simulink library "Simulation3DJoystickCalibratorLibrary"  (R2025b)
settings: Solver=VariableStepAuto  StartTime=0.0  StopTime=10.0  RelTol=1e-3
undefined symbols (not defined in the file or in its folder): aileronMax, aileronMin, elevatorMax, elevatorMin, helicopter, multirotor, pitchCh, pitchDB, pitchNeutral, rollCh, rollDB, rollNeutral, rudderMax, rudderMin, throttleCh, throttleDB, throttleMax, throttleMin, uPitchMax, uPitchMin, uRollMax, uRollMin, uThrottleMax, uThrottleMin, uYawMax, uYawMin, yawCh, yawDB, yawNeutral
libraries: sl3dlib x3
Description:
  | Simulation 3D Joystick Calibrator block library.
settings Model: Creator=klakhara  LastModifiedBy=klakhara

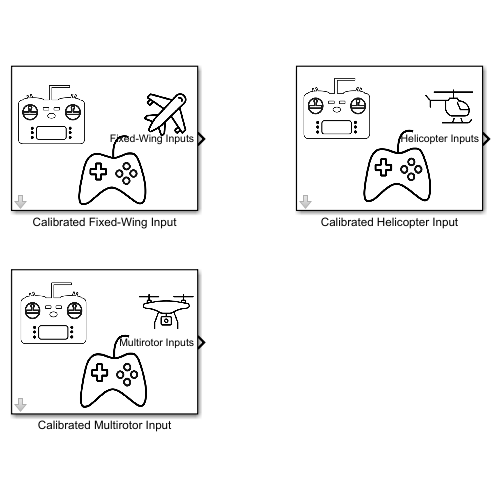
[thumbnail: Simulink's stored preview of the top-level diagram]
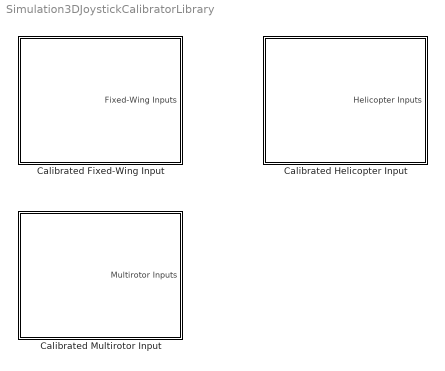
== system Simulation3DJoystickCalibratorLibrary ==
  Calibrated Fixed-Wing Input : Subsystem  mask{configName=0, joystickID=Joystick1, profileID=fixed-wing}
      mask prompts: joystickID "Device ID:"; profileID "Application profile"
      mask help: Calibrated Fixed-Wing Input. Accepts the shared Simulation 3D Joystick calibration. Output bus: Aileron, Elevator, Rudder, Throttle.
      mask TypeOptions joystickID: None | Joystick1 | Joystick2 | Joystick3 | Joystick4 | Joystick5 | Joystick6 | Joystick7 | Joystick8 | Joystick9 | Joystick10 | Joystick11 | Joystick12
      mask DialogControl DescGroupVar Prompt: Load Simulation 3D Joystick calibration
      mask DialogControl DescTextVar Prompt: Select a calibration configuration file:
      mask DialogControl loadConfig Prompt: Load file
      mask DialogControl openCalibrationApp Prompt: Open Calibration App
      mask DialogControl openCalibrationApp Tooltip: Open Simulation 3D Joystick Calibrator to create a calibration file.
      mask DialogControl ParameterGroupVar Prompt: Select the Simulation 3D Joystick device:
      mask Display: image('Calibrated Fixed Wing Aircraft Input.png');
  Calibrated Helicopter Input : Subsystem  mask{configName=0, joystickID=Joystick1, profileID=helicopter}
      mask prompts: joystickID "Device ID:"; profileID "Application profile"
      mask help: Calibrated Helicopter Input. Accepts the shared Simulation 3D Joystick calibration. Output bus: LateralCyclic, LongitudinalCyclic, Pedals, Collective.
      mask TypeOptions joystickID: None | Joystick1 | Joystick2 | Joystick3 | Joystick4 | Joystick5 | Joystick6 | Joystick7 | Joystick8 | Joystick9 | Joystick10 | Joystick11 | Joystick12
      mask DialogControl DescGroupVar Prompt: Load Simulation 3D Joystick calibration
      mask DialogControl DescTextVar Prompt: Select a calibration configuration file:
      mask DialogControl loadConfig Prompt: Load file
      mask DialogControl openCalibrationApp Prompt: Open Calibration App
      mask DialogControl openCalibrationApp Tooltip: Open Simulation 3D Joystick Calibrator to create a calibration file.
      mask DialogControl ParameterGroupVar Prompt: Select the Simulation 3D Joystick device:
      mask Display: image('Calibrated Helicopter Input.png');
  Calibrated Multirotor Input : Subsystem  mask{configName=0, joystickID=Joystick1, profileID=multirotor}
      mask prompts: joystickID "Device ID:"; profileID "Application profile"
      mask help: Calibrated Multirotor Input. Accepts the shared Simulation 3D Joystick calibration. Output bus: RollCmd, PitchCmd, YawCmd, ThrottleCmd.
      mask TypeOptions joystickID: None | Joystick1 | Joystick2 | Joystick3 | Joystick4 | Joystick5 | Joystick6 | Joystick7 | Joystick8 | Joystick9 | Joystick10 | Joystick11 | Joystick12
      mask DialogControl DescGroupVar Prompt: Load Simulation 3D Joystick calibration
      mask DialogControl DescTextVar Prompt: Select a calibration configuration file:
      mask DialogControl loadConfig Prompt: Load file
      mask DialogControl openCalibrationApp Prompt: Open Calibration App
      mask DialogControl openCalibrationApp Tooltip: Open Simulation 3D Joystick Calibrator to create a calibration file.
      mask DialogControl ParameterGroupVar Prompt: Select the Simulation 3D Joystick device:
      mask Display: image('Calibrated Rotorcraft Input.png');

== system Simulation3DJoystickCalibratorLibrary/Calibrated Fixed-Wing Input ==
  Actuator scaling : Subsystem
  CalibratedJoystickInput : BusCreator  Inputs=4
  Simulation 3D Joystick : sl3dlib/Simulation 3D/Hardware Interface/Simulation 3D Joystick  joyid=1  adjustports=on  forcefeed=off
  Terminator : Terminator
  Fixed-Wing Inputs : Outport
  wires:
  Simulation 3D Joystick/1 -> Actuator scaling/1(Raw Inputs)  "Raw Inputs"
  Actuator scaling/2(Elevator) -> CalibratedJoystickInput/2  "Elevator"
  Simulation 3D Joystick/2 -> Terminator/1
  CalibratedJoystickInput/1 -> Fixed-Wing Inputs/1  "Actuator deflections"
  Actuator scaling/3(Rudder) -> CalibratedJoystickInput/3  "Rudder"
  Actuator scaling/4(Throttle) -> CalibratedJoystickInput/4  "Throttle"
  Actuator scaling/1(Aileron) -> CalibratedJoystickInput/1  "Aileron"

== system Simulation3DJoystickCalibratorLibrary/Calibrated Helicopter Input ==
  Actuator scaling : Subsystem
  CalibratedJoystickInput : BusCreator  Inputs=4
  Simulation 3D Joystick : sl3dlib/Simulation 3D/Hardware Interface/Simulation 3D Joystick  joyid=1  adjustports=on  forcefeed=off
  Terminator : Terminator
  Helicopter Inputs : Outport
  wires:
  Simulation 3D Joystick/1 -> Actuator scaling/1(Raw Inputs)  "Raw Inputs"
  Actuator scaling/2(LongitudinalCyclic) -> CalibratedJoystickInput/2  "LongitudinalCyclic"
  Simulation 3D Joystick/2 -> Terminator/1
  CalibratedJoystickInput/1 -> Helicopter Inputs/1  "Actuator deflections"
  Actuator scaling/3(Pedals) -> CalibratedJoystickInput/3  "Pedals"
  Actuator scaling/4(Collective) -> CalibratedJoystickInput/4  "Collective"
  Actuator scaling/1(LateralCyclic) -> CalibratedJoystickInput/1  "LateralCyclic"

== system Simulation3DJoystickCalibratorLibrary/Calibrated Multirotor Input ==
  Actuator scaling : Subsystem
  CalibratedJoystickInput : BusCreator  Inputs=4
  Simulation 3D Joystick : sl3dlib/Simulation 3D/Hardware Interface/Simulation 3D Joystick  joyid=1  adjustports=on  forcefeed=off
  Terminator : Terminator
  Multirotor Inputs : Outport
  wires:
  Simulation 3D Joystick/1 -> Actuator scaling/1(Raw Inputs)  "Raw Inputs"
  Actuator scaling/2(PitchCmd) -> CalibratedJoystickInput/2  "PitchCmd"
  Simulation 3D Joystick/2 -> Terminator/1
  CalibratedJoystickInput/1 -> Multirotor Inputs/1  "Actuator deflections"
  Actuator scaling/3(YawCmd) -> CalibratedJoystickInput/3  "YawCmd"
  Actuator scaling/4(ThrottleCmd) -> CalibratedJoystickInput/4  "ThrottleCmd"
  Actuator scaling/1(RollCmd) -> CalibratedJoystickInput/1  "RollCmd"

== system Simulation3DJoystickCalibratorLibrary/Calibrated Fixed-Wing Input/Actuator scaling ==
  Raw Inputs : Inport
  Aileron Scaling : Subsystem
  Demux : Demux
  Elevator Scaling : Subsystem
  Rudder Scaling : Subsystem
  Selector : Selector  InputPortWidth=5  IndexOptions=Index vector (dialog)  Indices=[rollCh pitchCh yawCh throttleCh]  OutputSizes=1
  Throttle Scaling : Subsystem
  Aileron : Outport
  Elevator : Outport  Port=2
  Rudder : Outport  Port=3
  Throttle : Outport  Port=4
  wires:
  Raw Inputs/1 -> Selector/1
  Rudder Scaling/1(actuator deflection) -> Rudder/1
  Demux/3 -> Rudder Scaling/1(raw signal)  "Yaw"
  Demux/1 -> Aileron Scaling/1(raw signal)  "roll"
  Selector/1 -> Demux/1
  Elevator Scaling/1(actuator deflection) -> Elevator/1
  Demux/4 -> Throttle Scaling/1(raw signal)  "Throttle"
  Demux/2 -> Elevator Scaling/1(raw signal)  "Pitch"
  Aileron Scaling/1(actuator deflection) -> Aileron/1
  Throttle Scaling/1(actuator deflection) -> Throttle/1

== system Simulation3DJoystickCalibratorLibrary/Calibrated Helicopter Input/Actuator scaling ==
  Raw Inputs : Inport
  Collective Scaling : Subsystem
  Demux : Demux
  LateralCyclic Scaling : Subsystem
  LongitudinalCyclic Scaling : Subsystem
  Pedals Scaling : Subsystem
  Selector : Selector  InputPortWidth=5  IndexOptions=Index vector (dialog)  Indices=[rollCh pitchCh yawCh throttleCh]  OutputSizes=1
  LateralCyclic : Outport
  LongitudinalCyclic : Outport  Port=2
  Pedals : Outport  Port=3
  Collective : Outport  Port=4
  wires:
  Raw Inputs/1 -> Selector/1
  Pedals Scaling/1(actuator deflection) -> Pedals/1
  Demux/3 -> Pedals Scaling/1(raw signal)  "Yaw"
  Demux/1 -> LateralCyclic Scaling/1(raw signal)  "roll"
  Selector/1 -> Demux/1
  LongitudinalCyclic Scaling/1(actuator deflection) -> LongitudinalCyclic/1
  Demux/4 -> Collective Scaling/1(raw signal)  "Throttle"
  Demux/2 -> LongitudinalCyclic Scaling/1(raw signal)  "Pitch"
  LateralCyclic Scaling/1(actuator deflection) -> LateralCyclic/1
  Collective Scaling/1(actuator deflection) -> Collective/1

== system Simulation3DJoystickCalibratorLibrary/Calibrated Multirotor Input/Actuator scaling ==
  Raw Inputs : Inport
  Demux : Demux
  PitchCmd Scaling : Subsystem
  RollCmd Scaling : Subsystem
  Selector : Selector  InputPortWidth=5  IndexOptions=Index vector (dialog)  Indices=[rollCh pitchCh yawCh throttleCh]  OutputSizes=1
  ThrottleCmd Scaling : Subsystem
  YawCmd Scaling : Subsystem
  RollCmd : Outport
  PitchCmd : Outport  Port=2
  YawCmd : Outport  Port=3
  ThrottleCmd : Outport  Port=4
  wires:
  Raw Inputs/1 -> Selector/1
  YawCmd Scaling/1(actuator deflection) -> YawCmd/1
  Demux/3 -> YawCmd Scaling/1(raw signal)  "Yaw"
  Demux/1 -> RollCmd Scaling/1(raw signal)  "roll"
  Selector/1 -> Demux/1
  PitchCmd Scaling/1(actuator deflection) -> PitchCmd/1
  Demux/4 -> ThrottleCmd Scaling/1(raw signal)  "Throttle"
  Demux/2 -> PitchCmd Scaling/1(raw signal)  "Pitch"
  RollCmd Scaling/1(actuator deflection) -> RollCmd/1
  ThrottleCmd Scaling/1(actuator deflection) -> ThrottleCmd/1

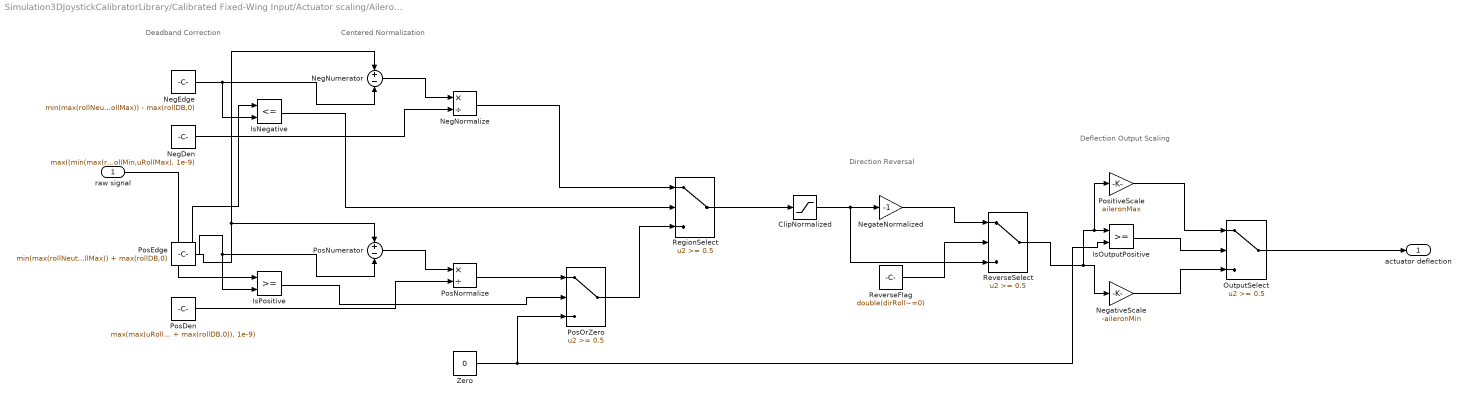
== system Simulation3DJoystickCalibratorLibrary/Calibrated Fixed-Wing Input/Actuator scaling/Aileron Scaling ==
  note: Deadband Correction
  note: Centered Normalization
  note: Direction Reversal
  note: Deflection Output Scaling
  raw signal : Inport
  ClipNormalized : Saturate  UpperLimit=1  LowerLimit=-1
  IsNegative : RelationalOperator  Operator=<=
  IsOutputPositive : RelationalOperator
  IsPositive : RelationalOperator
  NegDen : Constant  Value=max((min(max(rollNeutral,min(uRollMin,uRollMax)),max(uRollMin,uRollMax)) - max(rollDB,0)) - min(uRollMin,uRollMax), 1e-9)
  NegEdge : Constant  Value=min(max(rollNeutral,min(uRollMin,uRollMax)),max(uRollMin,uRollMax)) - max(rollDB,0)
  NegNormalize : Product  Inputs=*/
  NegNumerator : Sum  Inputs=+-
  NegateNormalized : Gain  Gain=-1
  NegativeScale : Gain  Gain=-aileronMin
  OutputSelect : Switch  Threshold=0.5
  PosDen : Constant  Value=max(max(uRollMin,uRollMax) - (min(max(rollNeutral,min(uRollMin,uRollMax)),max(uRollMin,uRollMax)) + max(rollDB,0)), 1e-9)
  PosEdge : Constant  Value=min(max(rollNeutral,min(uRollMin,uRollMax)),max(uRollMin,uRollMax)) + max(rollDB,0)
  PosNormalize : Product  Inputs=*/
  PosNumerator : Sum  Inputs=+-
  PosOrZero : Switch  Threshold=0.5
  PositiveScale : Gain  Gain=aileronMax
  RegionSelect : Switch  Threshold=0.5
  ReverseFlag : Constant  Value=double(dirRoll~=0)
  ReverseSelect : Switch  Threshold=0.5
  Zero : Constant  Value=0
  actuator deflection : Outport
  wires:
  raw signal/1 -> IsPositive/1, IsNegative/1, PosNumerator/1, NegNumerator/1
  NegEdge/1 -> IsNegative/2, NegNumerator/2
  NegNumerator/1 -> NegNormalize/1
  NegDen/1 -> NegNormalize/2
  PosEdge/1 -> IsPositive/2, PosNumerator/2
  PosNumerator/1 -> PosNormalize/1
  PosDen/1 -> PosNormalize/2
  PosNormalize/1 -> PosOrZero/1
  IsPositive/1 -> PosOrZero/2
  Zero/1 -> IsOutputPositive/2, PosOrZero/3
  NegNormalize/1 -> RegionSelect/1
  IsNegative/1 -> RegionSelect/2
  PosOrZero/1 -> RegionSelect/3
  RegionSelect/1 -> ClipNormalized/1
  ClipNormalized/1 -> ReverseSelect/3, NegateNormalized/1
  NegateNormalized/1 -> ReverseSelect/1
  ReverseFlag/1 -> ReverseSelect/2
  ReverseSelect/1 -> IsOutputPositive/1, PositiveScale/1, NegativeScale/1
  PositiveScale/1 -> OutputSelect/1
  IsOutputPositive/1 -> OutputSelect/2
  NegativeScale/1 -> OutputSelect/3
  OutputSelect/1 -> actuator deflection/1

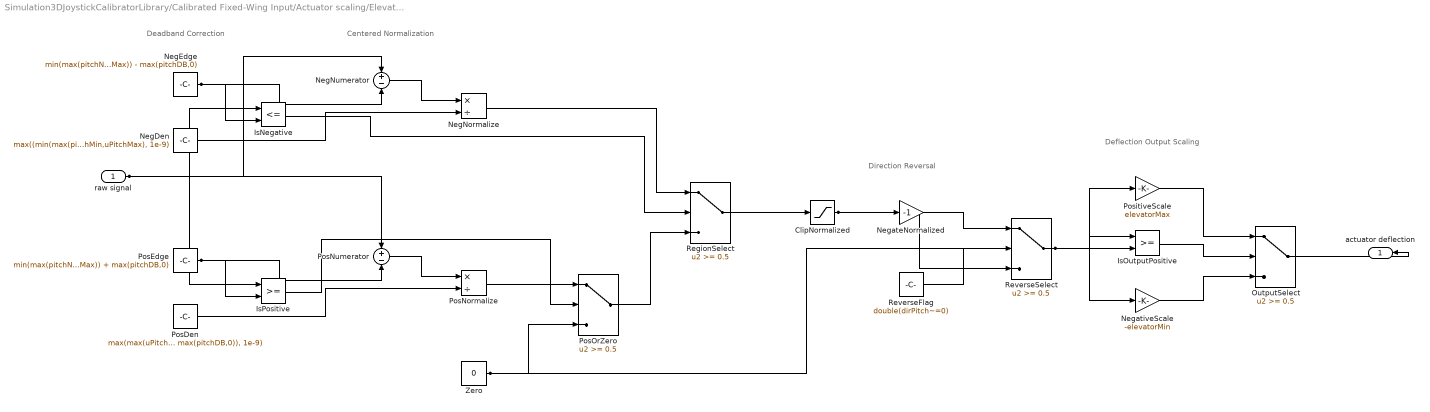
== system Simulation3DJoystickCalibratorLibrary/Calibrated Fixed-Wing Input/Actuator scaling/Elevator Scaling ==
  note: Deadband Correction
  note: Centered Normalization
  note: Direction Reversal
  note: Deflection Output Scaling
  raw signal : Inport
  ClipNormalized : Saturate  UpperLimit=1  LowerLimit=-1
  IsNegative : RelationalOperator  Operator=<=
  IsOutputPositive : RelationalOperator
  IsPositive : RelationalOperator
  NegDen : Constant  Value=max((min(max(pitchNeutral,min(uPitchMin,uPitchMax)),max(uPitchMin,uPitchMax)) - max(pitchDB,0)) - min(uPitchMin,uPitchMax), 1e-9)
  NegEdge : Constant  Value=min(max(pitchNeutral,min(uPitchMin,uPitchMax)),max(uPitchMin,uPitchMax)) - max(pitchDB,0)
  NegNormalize : Product  Inputs=*/
  NegNumerator : Sum  Inputs=+-
  NegateNormalized : Gain  Gain=-1
  NegativeScale : Gain  Gain=-elevatorMin
  OutputSelect : Switch  Threshold=0.5
  PosDen : Constant  Value=max(max(uPitchMin,uPitchMax) - (min(max(pitchNeutral,min(uPitchMin,uPitchMax)),max(uPitchMin,uPitchMax)) + max(pitchDB,0)), 1e-9)
  PosEdge : Constant  Value=min(max(pitchNeutral,min(uPitchMin,uPitchMax)),max(uPitchMin,uPitchMax)) + max(pitchDB,0)
  PosNormalize : Product  Inputs=*/
  PosNumerator : Sum  Inputs=+-
  PosOrZero : Switch  Threshold=0.5
  PositiveScale : Gain  Gain=elevatorMax
  RegionSelect : Switch  Threshold=0.5
  ReverseFlag : Constant  Value=double(dirPitch~=0)
  ReverseSelect : Switch  Threshold=0.5
  Zero : Constant  Value=0
  actuator deflection : Outport
  wires:
  raw signal/1 -> IsPositive/1, IsNegative/1, PosNumerator/1, NegNumerator/1
  NegEdge/1 -> IsNegative/2, NegNumerator/2
  NegNumerator/1 -> NegNormalize/1
  NegDen/1 -> NegNormalize/2
  PosEdge/1 -> IsPositive/2, PosNumerator/2
  PosNumerator/1 -> PosNormalize/1
  PosDen/1 -> PosNormalize/2
  PosNormalize/1 -> PosOrZero/1
  IsPositive/1 -> PosOrZero/2
  Zero/1 -> IsOutputPositive/2, PosOrZero/3
  NegNormalize/1 -> RegionSelect/1
  IsNegative/1 -> RegionSelect/2
  PosOrZero/1 -> RegionSelect/3
  RegionSelect/1 -> ClipNormalized/1
  ClipNormalized/1 -> ReverseSelect/3, NegateNormalized/1
  NegateNormalized/1 -> ReverseSelect/1
  ReverseFlag/1 -> ReverseSelect/2
  ReverseSelect/1 -> NegativeScale/1, PositiveScale/1, IsOutputPositive/1
  PositiveScale/1 -> OutputSelect/1
  IsOutputPositive/1 -> OutputSelect/2
  NegativeScale/1 -> OutputSelect/3
  OutputSelect/1 -> actuator deflection/1

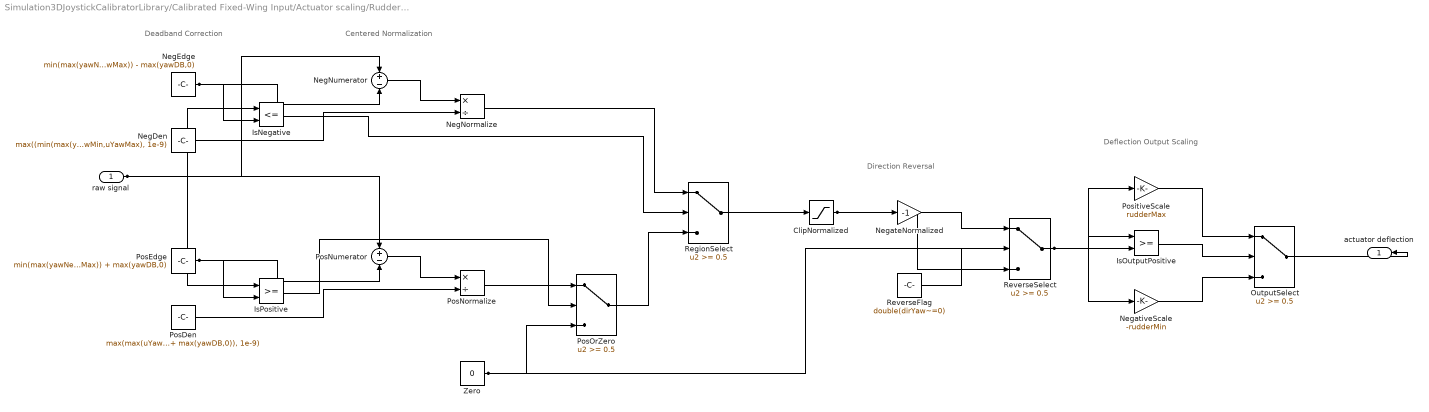
== system Simulation3DJoystickCalibratorLibrary/Calibrated Fixed-Wing Input/Actuator scaling/Rudder Scaling ==
  note: Deadband Correction
  note: Centered Normalization
  note: Direction Reversal
  note: Deflection Output Scaling
  raw signal : Inport
  ClipNormalized : Saturate  UpperLimit=1  LowerLimit=-1
  IsNegative : RelationalOperator  Operator=<=
  IsOutputPositive : RelationalOperator
  IsPositive : RelationalOperator
  NegDen : Constant  Value=max((min(max(yawNeutral,min(uYawMin,uYawMax)),max(uYawMin,uYawMax)) - max(yawDB,0)) - min(uYawMin,uYawMax), 1e-9)
  NegEdge : Constant  Value=min(max(yawNeutral,min(uYawMin,uYawMax)),max(uYawMin,uYawMax)) - max(yawDB,0)
  NegNormalize : Product  Inputs=*/
  NegNumerator : Sum  Inputs=+-
  NegateNormalized : Gain  Gain=-1
  NegativeScale : Gain  Gain=-rudderMin
  OutputSelect : Switch  Threshold=0.5
  PosDen : Constant  Value=max(max(uYawMin,uYawMax) - (min(max(yawNeutral,min(uYawMin,uYawMax)),max(uYawMin,uYawMax)) + max(yawDB,0)), 1e-9)
  PosEdge : Constant  Value=min(max(yawNeutral,min(uYawMin,uYawMax)),max(uYawMin,uYawMax)) + max(yawDB,0)
  PosNormalize : Product  Inputs=*/
  PosNumerator : Sum  Inputs=+-
  PosOrZero : Switch  Threshold=0.5
  PositiveScale : Gain  Gain=rudderMax
  RegionSelect : Switch  Threshold=0.5
  ReverseFlag : Constant  Value=double(dirYaw~=0)
  ReverseSelect : Switch  Threshold=0.5
  Zero : Constant  Value=0
  actuator deflection : Outport
  wires:
  raw signal/1 -> IsPositive/1, IsNegative/1, PosNumerator/1, NegNumerator/1
  NegEdge/1 -> IsNegative/2, NegNumerator/2
  NegNumerator/1 -> NegNormalize/1
  NegDen/1 -> NegNormalize/2
  PosEdge/1 -> IsPositive/2, PosNumerator/2
  PosNumerator/1 -> PosNormalize/1
  PosDen/1 -> PosNormalize/2
  PosNormalize/1 -> PosOrZero/1
  IsPositive/1 -> PosOrZero/2
  Zero/1 -> IsOutputPositive/2, PosOrZero/3
  NegNormalize/1 -> RegionSelect/1
  IsNegative/1 -> RegionSelect/2
  PosOrZero/1 -> RegionSelect/3
  RegionSelect/1 -> ClipNormalized/1
  ClipNormalized/1 -> ReverseSelect/3, NegateNormalized/1
  NegateNormalized/1 -> ReverseSelect/1
  ReverseFlag/1 -> ReverseSelect/2
  ReverseSelect/1 -> NegativeScale/1, PositiveScale/1, IsOutputPositive/1
  PositiveScale/1 -> OutputSelect/1
  IsOutputPositive/1 -> OutputSelect/2
  NegativeScale/1 -> OutputSelect/3
  OutputSelect/1 -> actuator deflection/1

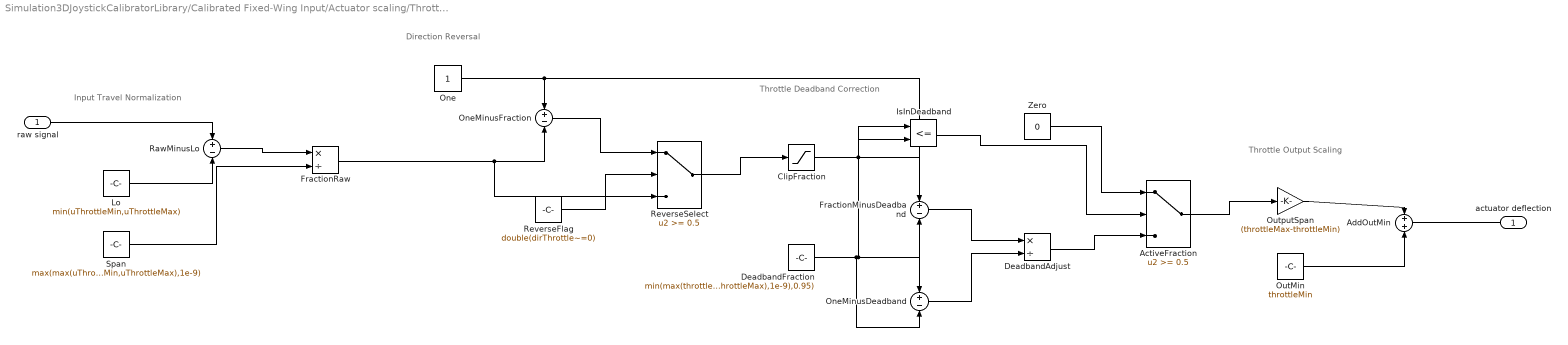
== system Simulation3DJoystickCalibratorLibrary/Calibrated Fixed-Wing Input/Actuator scaling/Throttle Scaling ==
  note: Input Travel Normalization
  note: Direction Reversal
  note: Throttle Deadband Correction
  note: Throttle Output Scaling
  raw signal : Inport
  ActiveFraction : Switch  Threshold=0.5
  AddOutMin : Sum
  ClipFraction : Saturate  UpperLimit=1  LowerLimit=0
  DeadbandAdjust : Product  Inputs=*/
  DeadbandFraction : Constant  Value=min(max(throttleDB,0)/max(max(uThrottleMin,uThrottleMax)-min(uThrottleMin,uThrottleMax),1e-9),0.95)
  FractionMinusDeadband : Sum  Inputs=+-
  FractionRaw : Product  Inputs=*/
  IsInDeadband : RelationalOperator  Operator=<=
  Lo : Constant  Value=min(uThrottleMin,uThrottleMax)
  One : Constant
  OneMinusDeadband : Sum  Inputs=+-
  OneMinusFraction : Sum  Inputs=+-
  OutMin : Constant  Value=throttleMin
  OutputSpan : Gain  Gain=(throttleMax-throttleMin)
  RawMinusLo : Sum  Inputs=+-
  ReverseFlag : Constant  Value=double(dirThrottle~=0)
  ReverseSelect : Switch  Threshold=0.5
  Span : Constant  Value=max(max(uThrottleMin,uThrottleMax)-min(uThrottleMin,uThrottleMax),1e-9)
  Zero : Constant  Value=0
  actuator deflection : Outport
  wires:
  raw signal/1 -> RawMinusLo/1
  Lo/1 -> RawMinusLo/2
  RawMinusLo/1 -> FractionRaw/1
  Span/1 -> FractionRaw/2
  One/1 -> OneMinusDeadband/1, OneMinusFraction/1
  FractionRaw/1 -> ReverseSelect/3, OneMinusFraction/2
  OneMinusFraction/1 -> ReverseSelect/1
  ReverseFlag/1 -> ReverseSelect/2
  ReverseSelect/1 -> ClipFraction/1
  ClipFraction/1 -> FractionMinusDeadband/1, IsInDeadband/1
  DeadbandFraction/1 -> OneMinusDeadband/2, FractionMinusDeadband/2, IsInDeadband/2
  FractionMinusDeadband/1 -> DeadbandAdjust/1
  OneMinusDeadband/1 -> DeadbandAdjust/2
  Zero/1 -> ActiveFraction/1
  IsInDeadband/1 -> ActiveFraction/2
  DeadbandAdjust/1 -> ActiveFraction/3
  ActiveFraction/1 -> OutputSpan/1
  OutputSpan/1 -> AddOutMin/1
  OutMin/1 -> AddOutMin/2
  AddOutMin/1 -> actuator deflection/1

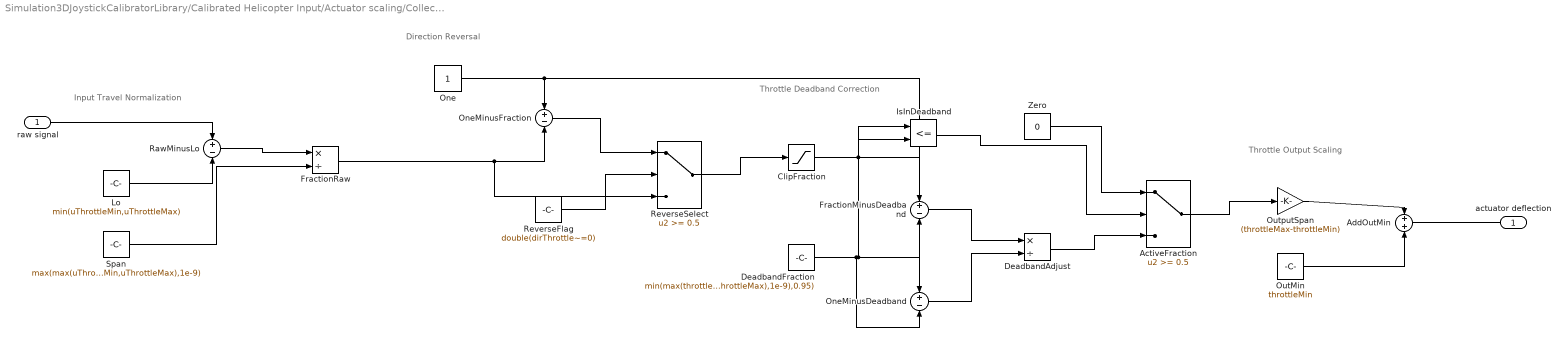
== system Simulation3DJoystickCalibratorLibrary/Calibrated Helicopter Input/Actuator scaling/Collective Scaling ==
  note: Input Travel Normalization
  note: Direction Reversal
  note: Throttle Deadband Correction
  note: Throttle Output Scaling
  raw signal : Inport
  ActiveFraction : Switch  Threshold=0.5
  AddOutMin : Sum
  ClipFraction : Saturate  UpperLimit=1  LowerLimit=0
  DeadbandAdjust : Product  Inputs=*/
  DeadbandFraction : Constant  Value=min(max(throttleDB,0)/max(max(uThrottleMin,uThrottleMax)-min(uThrottleMin,uThrottleMax),1e-9),0.95)
  FractionMinusDeadband : Sum  Inputs=+-
  FractionRaw : Product  Inputs=*/
  IsInDeadband : RelationalOperator  Operator=<=
  Lo : Constant  Value=min(uThrottleMin,uThrottleMax)
  One : Constant
  OneMinusDeadband : Sum  Inputs=+-
  OneMinusFraction : Sum  Inputs=+-
  OutMin : Constant  Value=throttleMin
  OutputSpan : Gain  Gain=(throttleMax-throttleMin)
  RawMinusLo : Sum  Inputs=+-
  ReverseFlag : Constant  Value=double(dirThrottle~=0)
  ReverseSelect : Switch  Threshold=0.5
  Span : Constant  Value=max(max(uThrottleMin,uThrottleMax)-min(uThrottleMin,uThrottleMax),1e-9)
  Zero : Constant  Value=0
  actuator deflection : Outport
  wires:
  raw signal/1 -> RawMinusLo/1
  Lo/1 -> RawMinusLo/2
  RawMinusLo/1 -> FractionRaw/1
  Span/1 -> FractionRaw/2
  One/1 -> OneMinusDeadband/1, OneMinusFraction/1
  FractionRaw/1 -> ReverseSelect/3, OneMinusFraction/2
  OneMinusFraction/1 -> ReverseSelect/1
  ReverseFlag/1 -> ReverseSelect/2
  ReverseSelect/1 -> ClipFraction/1
  ClipFraction/1 -> FractionMinusDeadband/1, IsInDeadband/1
  DeadbandFraction/1 -> OneMinusDeadband/2, FractionMinusDeadband/2, IsInDeadband/2
  FractionMinusDeadband/1 -> DeadbandAdjust/1
  OneMinusDeadband/1 -> DeadbandAdjust/2
  Zero/1 -> ActiveFraction/1
  IsInDeadband/1 -> ActiveFraction/2
  DeadbandAdjust/1 -> ActiveFraction/3
  ActiveFraction/1 -> OutputSpan/1
  OutputSpan/1 -> AddOutMin/1
  OutMin/1 -> AddOutMin/2
  AddOutMin/1 -> actuator deflection/1

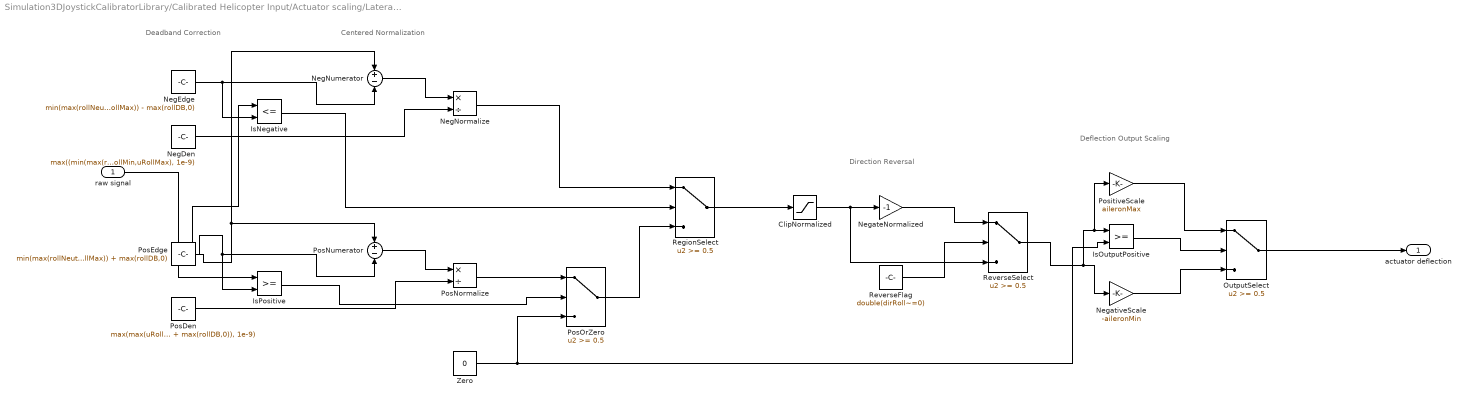
== system Simulation3DJoystickCalibratorLibrary/Calibrated Helicopter Input/Actuator scaling/LateralCyclic Scaling ==
  note: Deadband Correction
  note: Centered Normalization
  note: Direction Reversal
  note: Deflection Output Scaling
  raw signal : Inport
  ClipNormalized : Saturate  UpperLimit=1  LowerLimit=-1
  IsNegative : RelationalOperator  Operator=<=
  IsOutputPositive : RelationalOperator
  IsPositive : RelationalOperator
  NegDen : Constant  Value=max((min(max(rollNeutral,min(uRollMin,uRollMax)),max(uRollMin,uRollMax)) - max(rollDB,0)) - min(uRollMin,uRollMax), 1e-9)
  NegEdge : Constant  Value=min(max(rollNeutral,min(uRollMin,uRollMax)),max(uRollMin,uRollMax)) - max(rollDB,0)
  NegNormalize : Product  Inputs=*/
  NegNumerator : Sum  Inputs=+-
  NegateNormalized : Gain  Gain=-1
  NegativeScale : Gain  Gain=-aileronMin
  OutputSelect : Switch  Threshold=0.5
  PosDen : Constant  Value=max(max(uRollMin,uRollMax) - (min(max(rollNeutral,min(uRollMin,uRollMax)),max(uRollMin,uRollMax)) + max(rollDB,0)), 1e-9)
  PosEdge : Constant  Value=min(max(rollNeutral,min(uRollMin,uRollMax)),max(uRollMin,uRollMax)) + max(rollDB,0)
  PosNormalize : Product  Inputs=*/
  PosNumerator : Sum  Inputs=+-
  PosOrZero : Switch  Threshold=0.5
  PositiveScale : Gain  Gain=aileronMax
  RegionSelect : Switch  Threshold=0.5
  ReverseFlag : Constant  Value=double(dirRoll~=0)
  ReverseSelect : Switch  Threshold=0.5
  Zero : Constant  Value=0
  actuator deflection : Outport
  wires:
  raw signal/1 -> IsPositive/1, IsNegative/1, PosNumerator/1, NegNumerator/1
  NegEdge/1 -> IsNegative/2, NegNumerator/2
  NegNumerator/1 -> NegNormalize/1
  NegDen/1 -> NegNormalize/2
  PosEdge/1 -> IsPositive/2, PosNumerator/2
  PosNumerator/1 -> PosNormalize/1
  PosDen/1 -> PosNormalize/2
  PosNormalize/1 -> PosOrZero/1
  IsPositive/1 -> PosOrZero/2
  Zero/1 -> IsOutputPositive/2, PosOrZero/3
  NegNormalize/1 -> RegionSelect/1
  IsNegative/1 -> RegionSelect/2
  PosOrZero/1 -> RegionSelect/3
  RegionSelect/1 -> ClipNormalized/1
  ClipNormalized/1 -> ReverseSelect/3, NegateNormalized/1
  NegateNormalized/1 -> ReverseSelect/1
  ReverseFlag/1 -> ReverseSelect/2
  ReverseSelect/1 -> IsOutputPositive/1, PositiveScale/1, NegativeScale/1
  PositiveScale/1 -> OutputSelect/1
  IsOutputPositive/1 -> OutputSelect/2
  NegativeScale/1 -> OutputSelect/3
  OutputSelect/1 -> actuator deflection/1

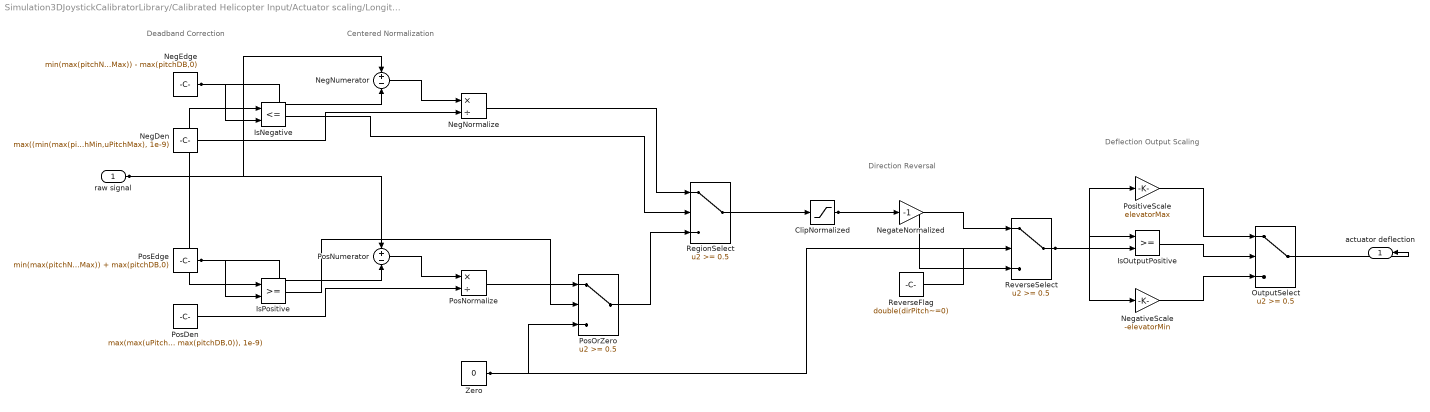
== system Simulation3DJoystickCalibratorLibrary/Calibrated Helicopter Input/Actuator scaling/LongitudinalCyclic Scaling ==
  note: Deadband Correction
  note: Centered Normalization
  note: Direction Reversal
  note: Deflection Output Scaling
  raw signal : Inport
  ClipNormalized : Saturate  UpperLimit=1  LowerLimit=-1
  IsNegative : RelationalOperator  Operator=<=
  IsOutputPositive : RelationalOperator
  IsPositive : RelationalOperator
  NegDen : Constant  Value=max((min(max(pitchNeutral,min(uPitchMin,uPitchMax)),max(uPitchMin,uPitchMax)) - max(pitchDB,0)) - min(uPitchMin,uPitchMax), 1e-9)
  NegEdge : Constant  Value=min(max(pitchNeutral,min(uPitchMin,uPitchMax)),max(uPitchMin,uPitchMax)) - max(pitchDB,0)
  NegNormalize : Product  Inputs=*/
  NegNumerator : Sum  Inputs=+-
  NegateNormalized : Gain  Gain=-1
  NegativeScale : Gain  Gain=-elevatorMin
  OutputSelect : Switch  Threshold=0.5
  PosDen : Constant  Value=max(max(uPitchMin,uPitchMax) - (min(max(pitchNeutral,min(uPitchMin,uPitchMax)),max(uPitchMin,uPitchMax)) + max(pitchDB,0)), 1e-9)
  PosEdge : Constant  Value=min(max(pitchNeutral,min(uPitchMin,uPitchMax)),max(uPitchMin,uPitchMax)) + max(pitchDB,0)
  PosNormalize : Product  Inputs=*/
  PosNumerator : Sum  Inputs=+-
  PosOrZero : Switch  Threshold=0.5
  PositiveScale : Gain  Gain=elevatorMax
  RegionSelect : Switch  Threshold=0.5
  ReverseFlag : Constant  Value=double(dirPitch~=0)
  ReverseSelect : Switch  Threshold=0.5
  Zero : Constant  Value=0
  actuator deflection : Outport
  wires:
  raw signal/1 -> IsPositive/1, IsNegative/1, PosNumerator/1, NegNumerator/1
  NegEdge/1 -> IsNegative/2, NegNumerator/2
  NegNumerator/1 -> NegNormalize/1
  NegDen/1 -> NegNormalize/2
  PosEdge/1 -> IsPositive/2, PosNumerator/2
  PosNumerator/1 -> PosNormalize/1
  PosDen/1 -> PosNormalize/2
  PosNormalize/1 -> PosOrZero/1
  IsPositive/1 -> PosOrZero/2
  Zero/1 -> IsOutputPositive/2, PosOrZero/3
  NegNormalize/1 -> RegionSelect/1
  IsNegative/1 -> RegionSelect/2
  PosOrZero/1 -> RegionSelect/3
  RegionSelect/1 -> ClipNormalized/1
  ClipNormalized/1 -> ReverseSelect/3, NegateNormalized/1
  NegateNormalized/1 -> ReverseSelect/1
  ReverseFlag/1 -> ReverseSelect/2
  ReverseSelect/1 -> NegativeScale/1, PositiveScale/1, IsOutputPositive/1
  PositiveScale/1 -> OutputSelect/1
  IsOutputPositive/1 -> OutputSelect/2
  NegativeScale/1 -> OutputSelect/3
  OutputSelect/1 -> actuator deflection/1

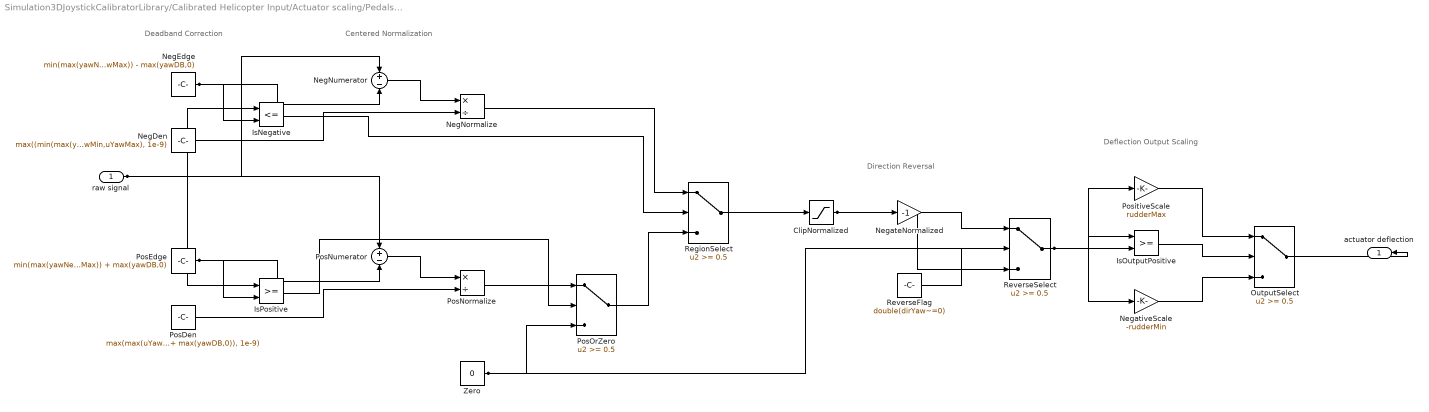
== system Simulation3DJoystickCalibratorLibrary/Calibrated Helicopter Input/Actuator scaling/Pedals Scaling ==
  note: Deadband Correction
  note: Centered Normalization
  note: Direction Reversal
  note: Deflection Output Scaling
  raw signal : Inport
  ClipNormalized : Saturate  UpperLimit=1  LowerLimit=-1
  IsNegative : RelationalOperator  Operator=<=
  IsOutputPositive : RelationalOperator
  IsPositive : RelationalOperator
  NegDen : Constant  Value=max((min(max(yawNeutral,min(uYawMin,uYawMax)),max(uYawMin,uYawMax)) - max(yawDB,0)) - min(uYawMin,uYawMax), 1e-9)
  NegEdge : Constant  Value=min(max(yawNeutral,min(uYawMin,uYawMax)),max(uYawMin,uYawMax)) - max(yawDB,0)
  NegNormalize : Product  Inputs=*/
  NegNumerator : Sum  Inputs=+-
  NegateNormalized : Gain  Gain=-1
  NegativeScale : Gain  Gain=-rudderMin
  OutputSelect : Switch  Threshold=0.5
  PosDen : Constant  Value=max(max(uYawMin,uYawMax) - (min(max(yawNeutral,min(uYawMin,uYawMax)),max(uYawMin,uYawMax)) + max(yawDB,0)), 1e-9)
  PosEdge : Constant  Value=min(max(yawNeutral,min(uYawMin,uYawMax)),max(uYawMin,uYawMax)) + max(yawDB,0)
  PosNormalize : Product  Inputs=*/
  PosNumerator : Sum  Inputs=+-
  PosOrZero : Switch  Threshold=0.5
  PositiveScale : Gain  Gain=rudderMax
  RegionSelect : Switch  Threshold=0.5
  ReverseFlag : Constant  Value=double(dirYaw~=0)
  ReverseSelect : Switch  Threshold=0.5
  Zero : Constant  Value=0
  actuator deflection : Outport
  wires:
  raw signal/1 -> IsPositive/1, IsNegative/1, PosNumerator/1, NegNumerator/1
  NegEdge/1 -> IsNegative/2, NegNumerator/2
  NegNumerator/1 -> NegNormalize/1
  NegDen/1 -> NegNormalize/2
  PosEdge/1 -> IsPositive/2, PosNumerator/2
  PosNumerator/1 -> PosNormalize/1
  PosDen/1 -> PosNormalize/2
  PosNormalize/1 -> PosOrZero/1
  IsPositive/1 -> PosOrZero/2
  Zero/1 -> IsOutputPositive/2, PosOrZero/3
  NegNormalize/1 -> RegionSelect/1
  IsNegative/1 -> RegionSelect/2
  PosOrZero/1 -> RegionSelect/3
  RegionSelect/1 -> ClipNormalized/1
  ClipNormalized/1 -> ReverseSelect/3, NegateNormalized/1
  NegateNormalized/1 -> ReverseSelect/1
  ReverseFlag/1 -> ReverseSelect/2
  ReverseSelect/1 -> NegativeScale/1, PositiveScale/1, IsOutputPositive/1
  PositiveScale/1 -> OutputSelect/1
  IsOutputPositive/1 -> OutputSelect/2
  NegativeScale/1 -> OutputSelect/3
  OutputSelect/1 -> actuator deflection/1

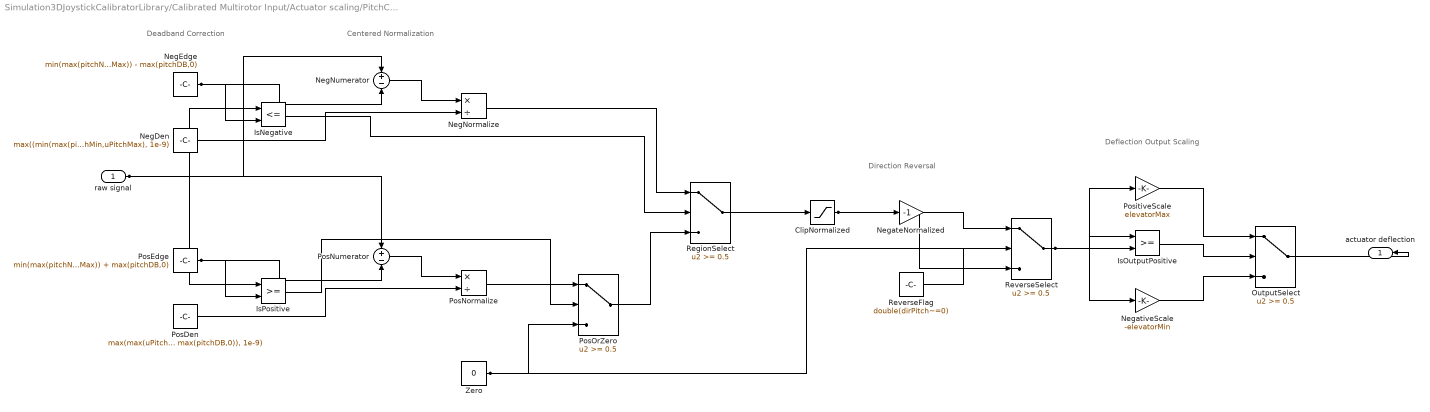
== system Simulation3DJoystickCalibratorLibrary/Calibrated Multirotor Input/Actuator scaling/PitchCmd Scaling ==
  note: Deadband Correction
  note: Centered Normalization
  note: Direction Reversal
  note: Deflection Output Scaling
  raw signal : Inport
  ClipNormalized : Saturate  UpperLimit=1  LowerLimit=-1
  IsNegative : RelationalOperator  Operator=<=
  IsOutputPositive : RelationalOperator
  IsPositive : RelationalOperator
  NegDen : Constant  Value=max((min(max(pitchNeutral,min(uPitchMin,uPitchMax)),max(uPitchMin,uPitchMax)) - max(pitchDB,0)) - min(uPitchMin,uPitchMax), 1e-9)
  NegEdge : Constant  Value=min(max(pitchNeutral,min(uPitchMin,uPitchMax)),max(uPitchMin,uPitchMax)) - max(pitchDB,0)
  NegNormalize : Product  Inputs=*/
  NegNumerator : Sum  Inputs=+-
  NegateNormalized : Gain  Gain=-1
  NegativeScale : Gain  Gain=-elevatorMin
  OutputSelect : Switch  Threshold=0.5
  PosDen : Constant  Value=max(max(uPitchMin,uPitchMax) - (min(max(pitchNeutral,min(uPitchMin,uPitchMax)),max(uPitchMin,uPitchMax)) + max(pitchDB,0)), 1e-9)
  PosEdge : Constant  Value=min(max(pitchNeutral,min(uPitchMin,uPitchMax)),max(uPitchMin,uPitchMax)) + max(pitchDB,0)
  PosNormalize : Product  Inputs=*/
  PosNumerator : Sum  Inputs=+-
  PosOrZero : Switch  Threshold=0.5
  PositiveScale : Gain  Gain=elevatorMax
  RegionSelect : Switch  Threshold=0.5
  ReverseFlag : Constant  Value=double(dirPitch~=0)
  ReverseSelect : Switch  Threshold=0.5
  Zero : Constant  Value=0
  actuator deflection : Outport
  wires:
  raw signal/1 -> IsPositive/1, IsNegative/1, PosNumerator/1, NegNumerator/1
  NegEdge/1 -> IsNegative/2, NegNumerator/2
  NegNumerator/1 -> NegNormalize/1
  NegDen/1 -> NegNormalize/2
  PosEdge/1 -> IsPositive/2, PosNumerator/2
  PosNumerator/1 -> PosNormalize/1
  PosDen/1 -> PosNormalize/2
  PosNormalize/1 -> PosOrZero/1
  IsPositive/1 -> PosOrZero/2
  Zero/1 -> IsOutputPositive/2, PosOrZero/3
  NegNormalize/1 -> RegionSelect/1
  IsNegative/1 -> RegionSelect/2
  PosOrZero/1 -> RegionSelect/3
  RegionSelect/1 -> ClipNormalized/1
  ClipNormalized/1 -> ReverseSelect/3, NegateNormalized/1
  NegateNormalized/1 -> ReverseSelect/1
  ReverseFlag/1 -> ReverseSelect/2
  ReverseSelect/1 -> NegativeScale/1, PositiveScale/1, IsOutputPositive/1
  PositiveScale/1 -> OutputSelect/1
  IsOutputPositive/1 -> OutputSelect/2
  NegativeScale/1 -> OutputSelect/3
  OutputSelect/1 -> actuator deflection/1

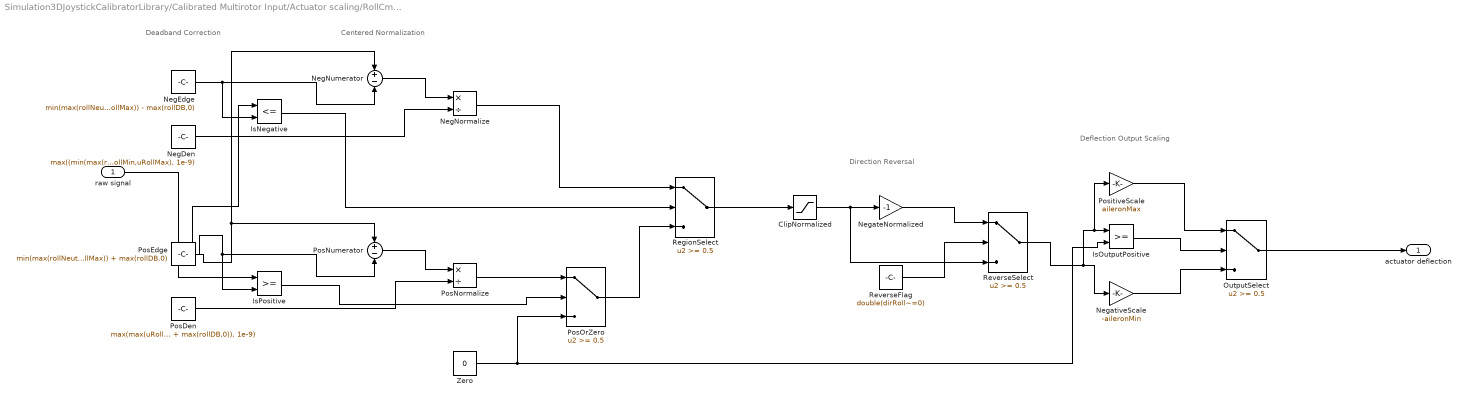
== system Simulation3DJoystickCalibratorLibrary/Calibrated Multirotor Input/Actuator scaling/RollCmd Scaling ==
  note: Deadband Correction
  note: Centered Normalization
  note: Direction Reversal
  note: Deflection Output Scaling
  raw signal : Inport
  ClipNormalized : Saturate  UpperLimit=1  LowerLimit=-1
  IsNegative : RelationalOperator  Operator=<=
  IsOutputPositive : RelationalOperator
  IsPositive : RelationalOperator
  NegDen : Constant  Value=max((min(max(rollNeutral,min(uRollMin,uRollMax)),max(uRollMin,uRollMax)) - max(rollDB,0)) - min(uRollMin,uRollMax), 1e-9)
  NegEdge : Constant  Value=min(max(rollNeutral,min(uRollMin,uRollMax)),max(uRollMin,uRollMax)) - max(rollDB,0)
  NegNormalize : Product  Inputs=*/
  NegNumerator : Sum  Inputs=+-
  NegateNormalized : Gain  Gain=-1
  NegativeScale : Gain  Gain=-aileronMin
  OutputSelect : Switch  Threshold=0.5
  PosDen : Constant  Value=max(max(uRollMin,uRollMax) - (min(max(rollNeutral,min(uRollMin,uRollMax)),max(uRollMin,uRollMax)) + max(rollDB,0)), 1e-9)
  PosEdge : Constant  Value=min(max(rollNeutral,min(uRollMin,uRollMax)),max(uRollMin,uRollMax)) + max(rollDB,0)
  PosNormalize : Product  Inputs=*/
  PosNumerator : Sum  Inputs=+-
  PosOrZero : Switch  Threshold=0.5
  PositiveScale : Gain  Gain=aileronMax
  RegionSelect : Switch  Threshold=0.5
  ReverseFlag : Constant  Value=double(dirRoll~=0)
  ReverseSelect : Switch  Threshold=0.5
  Zero : Constant  Value=0
  actuator deflection : Outport
  wires:
  raw signal/1 -> IsPositive/1, IsNegative/1, PosNumerator/1, NegNumerator/1
  NegEdge/1 -> IsNegative/2, NegNumerator/2
  NegNumerator/1 -> NegNormalize/1
  NegDen/1 -> NegNormalize/2
  PosEdge/1 -> IsPositive/2, PosNumerator/2
  PosNumerator/1 -> PosNormalize/1
  PosDen/1 -> PosNormalize/2
  PosNormalize/1 -> PosOrZero/1
  IsPositive/1 -> PosOrZero/2
  Zero/1 -> IsOutputPositive/2, PosOrZero/3
  NegNormalize/1 -> RegionSelect/1
  IsNegative/1 -> RegionSelect/2
  PosOrZero/1 -> RegionSelect/3
  RegionSelect/1 -> ClipNormalized/1
  ClipNormalized/1 -> ReverseSelect/3, NegateNormalized/1
  NegateNormalized/1 -> ReverseSelect/1
  ReverseFlag/1 -> ReverseSelect/2
  ReverseSelect/1 -> IsOutputPositive/1, PositiveScale/1, NegativeScale/1
  PositiveScale/1 -> OutputSelect/1
  IsOutputPositive/1 -> OutputSelect/2
  NegativeScale/1 -> OutputSelect/3
  OutputSelect/1 -> actuator deflection/1

== system Simulation3DJoystickCalibratorLibrary/Calibrated Multirotor Input/Actuator scaling/ThrottleCmd Scaling ==
  note: Input Travel Normalization
  note: Direction Reversal
  note: Throttle Deadband Correction
  note: Throttle Output Scaling
  raw signal : Inport
  ActiveFraction : Switch  Threshold=0.5
  AddOutMin : Sum
  ClipFraction : Saturate  UpperLimit=1  LowerLimit=0
  DeadbandAdjust : Product  Inputs=*/
  DeadbandFraction : Constant  Value=min(max(throttleDB,0)/max(max(uThrottleMin,uThrottleMax)-min(uThrottleMin,uThrottleMax),1e-9),0.95)
  FractionMinusDeadband : Sum  Inputs=+-
  FractionRaw : Product  Inputs=*/
  IsInDeadband : RelationalOperator  Operator=<=
  Lo : Constant  Value=min(uThrottleMin,uThrottleMax)
  One : Constant
  OneMinusDeadband : Sum  Inputs=+-
  OneMinusFraction : Sum  Inputs=+-
  OutMin : Constant  Value=throttleMin
  OutputSpan : Gain  Gain=(throttleMax-throttleMin)
  RawMinusLo : Sum  Inputs=+-
  ReverseFlag : Constant  Value=double(dirThrottle~=0)
  ReverseSelect : Switch  Threshold=0.5
  Span : Constant  Value=max(max(uThrottleMin,uThrottleMax)-min(uThrottleMin,uThrottleMax),1e-9)
  Zero : Constant  Value=0
  actuator deflection : Outport
  wires:
  raw signal/1 -> RawMinusLo/1
  Lo/1 -> RawMinusLo/2
  RawMinusLo/1 -> FractionRaw/1
  Span/1 -> FractionRaw/2
  One/1 -> OneMinusDeadband/1, OneMinusFraction/1
  FractionRaw/1 -> ReverseSelect/3, OneMinusFraction/2
  OneMinusFraction/1 -> ReverseSelect/1
  ReverseFlag/1 -> ReverseSelect/2
  ReverseSelect/1 -> ClipFraction/1
  ClipFraction/1 -> FractionMinusDeadband/1, IsInDeadband/1
  DeadbandFraction/1 -> OneMinusDeadband/2, FractionMinusDeadband/2, IsInDeadband/2
  FractionMinusDeadband/1 -> DeadbandAdjust/1
  OneMinusDeadband/1 -> DeadbandAdjust/2
  Zero/1 -> ActiveFraction/1
  IsInDeadband/1 -> ActiveFraction/2
  DeadbandAdjust/1 -> ActiveFraction/3
  ActiveFraction/1 -> OutputSpan/1
  OutputSpan/1 -> AddOutMin/1
  OutMin/1 -> AddOutMin/2
  AddOutMin/1 -> actuator deflection/1

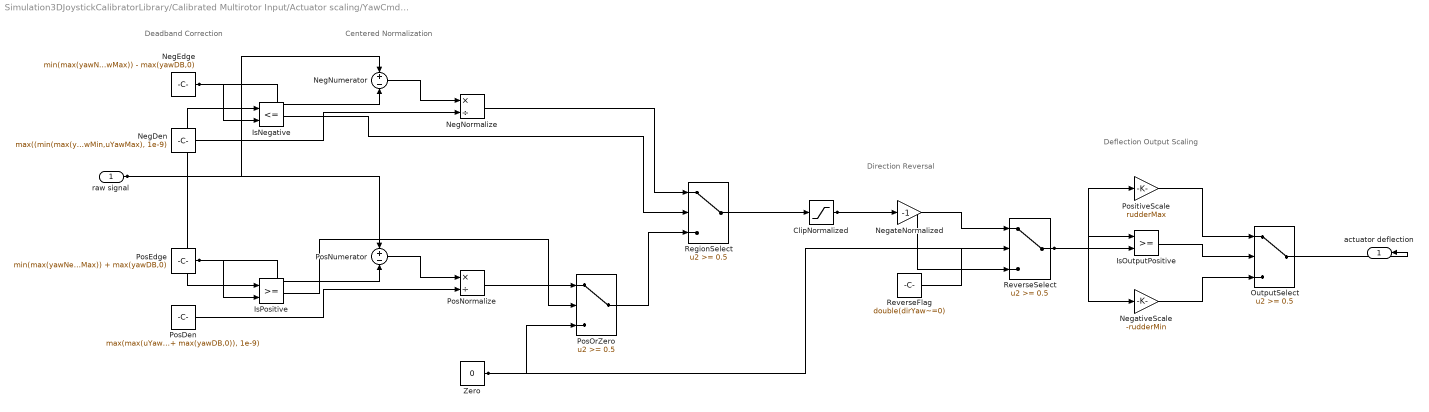
== system Simulation3DJoystickCalibratorLibrary/Calibrated Multirotor Input/Actuator scaling/YawCmd Scaling ==
  note: Deadband Correction
  note: Centered Normalization
  note: Direction Reversal
  note: Deflection Output Scaling
  raw signal : Inport
  ClipNormalized : Saturate  UpperLimit=1  LowerLimit=-1
  IsNegative : RelationalOperator  Operator=<=
  IsOutputPositive : RelationalOperator
  IsPositive : RelationalOperator
  NegDen : Constant  Value=max((min(max(yawNeutral,min(uYawMin,uYawMax)),max(uYawMin,uYawMax)) - max(yawDB,0)) - min(uYawMin,uYawMax), 1e-9)
  NegEdge : Constant  Value=min(max(yawNeutral,min(uYawMin,uYawMax)),max(uYawMin,uYawMax)) - max(yawDB,0)
  NegNormalize : Product  Inputs=*/
  NegNumerator : Sum  Inputs=+-
  NegateNormalized : Gain  Gain=-1
  NegativeScale : Gain  Gain=-rudderMin
  OutputSelect : Switch  Threshold=0.5
  PosDen : Constant  Value=max(max(uYawMin,uYawMax) - (min(max(yawNeutral,min(uYawMin,uYawMax)),max(uYawMin,uYawMax)) + max(yawDB,0)), 1e-9)
  PosEdge : Constant  Value=min(max(yawNeutral,min(uYawMin,uYawMax)),max(uYawMin,uYawMax)) + max(yawDB,0)
  PosNormalize : Product  Inputs=*/
  PosNumerator : Sum  Inputs=+-
  PosOrZero : Switch  Threshold=0.5
  PositiveScale : Gain  Gain=rudderMax
  RegionSelect : Switch  Threshold=0.5
  ReverseFlag : Constant  Value=double(dirYaw~=0)
  ReverseSelect : Switch  Threshold=0.5
  Zero : Constant  Value=0
  actuator deflection : Outport
  wires:
  raw signal/1 -> IsPositive/1, IsNegative/1, PosNumerator/1, NegNumerator/1
  NegEdge/1 -> IsNegative/2, NegNumerator/2
  NegNumerator/1 -> NegNormalize/1
  NegDen/1 -> NegNormalize/2
  PosEdge/1 -> IsPositive/2, PosNumerator/2
  PosNumerator/1 -> PosNormalize/1
  PosDen/1 -> PosNormalize/2
  PosNormalize/1 -> PosOrZero/1
  IsPositive/1 -> PosOrZero/2
  Zero/1 -> IsOutputPositive/2, PosOrZero/3
  NegNormalize/1 -> RegionSelect/1
  IsNegative/1 -> RegionSelect/2
  PosOrZero/1 -> RegionSelect/3
  RegionSelect/1 -> ClipNormalized/1
  ClipNormalized/1 -> ReverseSelect/3, NegateNormalized/1
  NegateNormalized/1 -> ReverseSelect/1
  ReverseFlag/1 -> ReverseSelect/2
  ReverseSelect/1 -> NegativeScale/1, PositiveScale/1, IsOutputPositive/1
  PositiveScale/1 -> OutputSelect/1
  IsOutputPositive/1 -> OutputSelect/2
  NegativeScale/1 -> OutputSelect/3
  OutputSelect/1 -> actuator deflection/1
